simulink model "Chapter6"  (R2024b)
settings: Solver=ode4  StartTime=0.0  StopTime=SIM.StopTime  FixedStep=SIM.FixedStepSize  RelTol=1e-3
values from neighbouring files (symbols this model uses):
  AP = computeAutopilotGains(MAV, TRIM, TFS, DES)    [ch6_main.m]    (also in computeAutopilotGains.m = struct())
  CMD = struct()    [ch6_main.m]
  DES = loadDesignParams()    [ch6_main.m]    (also in loadDesignParams.m = struct())
  LIM = loadSafetyLimits()    [ch6_main.m]
  TRIM =     [ch6.mat]    (also in ch6_main.m = findTrim(TRIM_MODEL, Va_trim, R_trim, gamma_trim, TRIM_DATA_; findTrim.m = struct())
undefined symbols (not defined in the file or in its folder): drawAircraft, MAV, plotter, SIM
libraries: simulink x8, matrix_library x2
(part 2 of 2)

== matlab function Chapter6/Plant/Subsystem1/Subsystem/MATLAB Function ==
  data: u input; y output
function y = fcn(u)
    sphi = sin(u(1));
    cphi = cos(u(1));

    sthe = sin(u(2));
    cthe = cos(u(2));

    scthe = 1 / cthe;
    tthe = scthe * sthe;

    y = [1 sphi * tthe cphi*tthe;
         0 cphi -sphi;
         0 sphi*scthe cphi*scthe];

== matlab function Chapter6/Autopilot/Lateral Autopilot/Sideslip Hold Control Loop/MATLAB Function ==
  data: u_unsat input; I output; u_sat input; Ki_e input
function I = clampAntiWindup(u_unsat, u_sat, Ki_e)
    is_saturated = (u_unsat ~= u_sat);
    is_same_dir = (u_unsat * Ki_e > 0);

    if (is_saturated && is_same_dir), I = 0;
    else, I = Ki_e;
    end
end

== matlab function Chapter6/Autopilot/Lateral Autopilot/Course Hold Control Loop/MATLAB Function ==
  data: u_unsat input; I output; u_sat input; Ki_e input
function I = clampAntiWindup(u_unsat, u_sat, Ki_e)
    is_saturated = (u_unsat ~= u_sat);
    is_same_dir = (u_unsat * Ki_e > 0);

    if (is_saturated && is_same_dir), I = 0;
    else, I = Ki_e;
    end
end

== matlab function Chapter6/Autopilot/Lateral Autopilot/Course Hold Control Loop/Roll Hold Control Loop/MATLAB Function ==
  data: u_unsat input; I output; u_sat input; Ki_e input
function I = clampAntiWindup(u_unsat, u_sat, Ki_e)
    is_saturated = (u_unsat ~= u_sat);
    is_same_dir = (u_unsat * Ki_e > 0);

    if (is_saturated && is_same_dir), I = 0;
    else, I = Ki_e;
    end
end

== matlab function Chapter6/Autopilot/Longitudinal Autopilot/Altitude Hold Control Outer Loop/MATLAB Function ==
  data: u_unsat input; I output; u_sat input; Ki_e input
function I = clampAntiWindup(u_unsat, u_sat, Ki_e)
    is_saturated = (u_unsat ~= u_sat);
    is_same_dir = (u_unsat * Ki_e > 0);

    if (is_saturated && is_same_dir), I = 0;
    else, I = Ki_e;
    end
end

== matlab function Chapter6/Autopilot/Longitudinal Autopilot/Airspeed Hold Control using Pitch Outer Loop/MATLAB Function ==
  data: u_unsat input; I output; u_sat input; Ki_e input
function I = clampAntiWindup(u_unsat, u_sat, Ki_e)
    is_saturated = (u_unsat ~= u_sat);
    is_same_dir = (u_unsat * Ki_e > 0);

    if (is_saturated && is_same_dir), I = 0;
    else, I = Ki_e;
    end
end

== matlab function Chapter6/Autopilot/Longitudinal Autopilot/Airspeed Hold Control using Throttle /MATLAB Function ==
  data: u_unsat input; I output; u_sat input; Ki_e input
function I = clampAntiWindup(u_unsat, u_sat, Ki_e)
    is_saturated = (u_unsat ~= u_sat);
    is_same_dir = (u_unsat * Ki_e > 0);

    if (is_saturated && is_same_dir), I = 0;
    else, I = Ki_e;
    end
end
